simulink model "stm1"  (Simulink 5.0)
settings: Solver=ode45  StartTime=0.0  StopTime=100  RelTol=1e-3
undefined symbols (not defined in the file): F, I
settings Model: Creator=mcarroll  LastModifiedBy=mcarroll  ExtModeAutoUpdateStatusClock=off  OptimizeBlockIOStorage=off

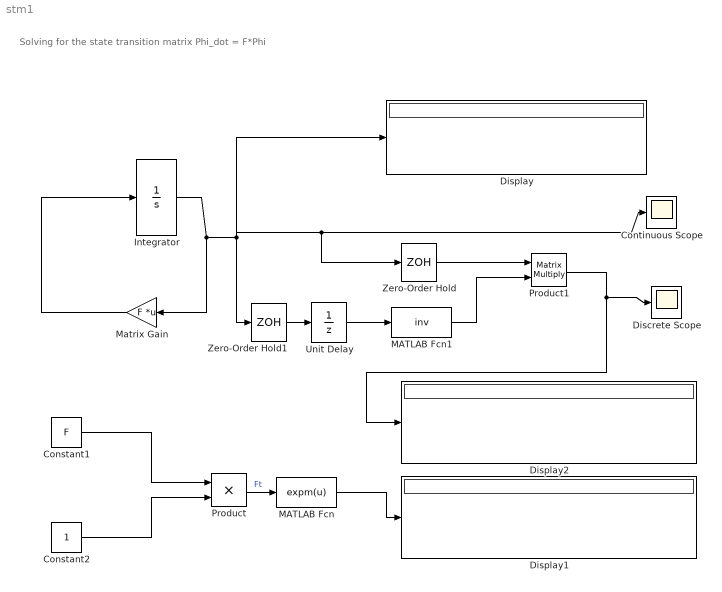
== system stm1 ==
  note: Solving for the state transition matrix
      | Phi_dot = F*Phi
  Constant1 : Constant  Value=F
  Constant2 : Constant
  Continuous Scope : Scope
  Discrete Scope : Scope
  Display : Display
  Display1 : Display
  Display2 : Display
  Integrator : Integrator  InitialCondition=I
  MATLAB Fcn : MATLABFcn  MATLABFcn=expm(u)  Output1D=off
  MATLAB Fcn1 : MATLABFcn  MATLABFcn=inv  Output1D=off
  Matrix Gain : Gain  Orientation=left  Gain=F  Multiplication=Matrix(K*u)  SaturateOnIntegerOverflow=on
  Product : Product  SaturateOnIntegerOverflow=on  InputSameDT=on
  Product1 : Product  Multiplication=Matrix(*)  SaturateOnIntegerOverflow=on  InputSameDT=on
  Unit Delay : UnitDelay  X0=I
  Zero-Order Hold : ZeroOrderHold
  Zero-Order Hold1 : ZeroOrderHold
  wires:
  Integrator/1 -> Display/1, Continuous Scope/1, Zero-Order Hold/1, Zero-Order Hold1/1, Matrix Gain/1
  Matrix Gain/1 -> Integrator/1
  Constant2/1 -> Product/2
  Product/1 -> MATLAB Fcn/1  "Ft"
  Constant1/1 -> Product/1
  MATLAB Fcn/1 -> Display1/1
  Unit Delay/1 -> MATLAB Fcn1/1
  MATLAB Fcn1/1 -> Product1/2
  Product1/1 -> Discrete Scope/1, Display2/1
  Zero-Order Hold/1 -> Product1/1
  Zero-Order Hold1/1 -> Unit Delay/1
